simulink library "Scissor_Parts_Lib"  (R2025a)
settings: Solver=ode45  StartTime=0.0  StopTime=10.0  RelTol=1e-3  EnableMultiTasking=on
undefined symbols (not defined in the file or in its folder): Extr_Data_LinkHoles, Extr_Data_Ring, Local, Scissor_Lift_Param, X, Y, Z
libraries: sm_lib x23, $bdroot x16
Description:
  | Copyright 2015-2025 The MathWorks, Inc.
settings Model: Creator=smiller  LastModifiedBy=smiller
settings SolverCC: AlgebraicLoopSolver=TrustRegion
settings DataIOCC: LimitDataPoints=on  SaveFormat=Array  SignalLoggingSaveFormat=ModelDataLogs  ReturnWorkspaceOutputs=off
settings OptimizationCC: ReuseModelBlockBuffer=off  ExpressionDepthLimit=2147483647.0  LifeSpan=inf
settings DebuggingCC: UnderspecifiedInitializationDetection=Classic  MergeDetectMultiDrivingBlocksExec=none  SolverPrmCheckMsg=warning  FcnCallInpInsideContextMsg=warning  UnconnectedInputMsg=warning  UnconnectedOutputMsg=warning  UnconnectedLineMsg=warning  AllowSymbolicDim=off  StateNameClashWarn=warning  PregeneratedLibrarySubsystemCodeDiagnostic=none  SFUnexpectedBacktrackingDiag=warning  SFNoUnconditionalDefaultTransitionDiag=warning  SFExecutionAtInitializationDiag=none  ArithmeticOperatorsInVariantConditions=warning
settings HardwareCC: ProdBitPerPointer=32.0  ProdBitPerSizeT=32.0  ProdBitPerPtrDiffT=32.0  ProdLargestAtomicFloat=None  ProdIntDivRoundTo=Undefined  ProdEndianess=Unspecified  ProdWordSize=32.0  ProdHWDeviceType=32-bit Generic
settings ModelReferenceCC: EnableRefExpFcnMdlSchedulingChecks=on  PropagateSignalLabelsOutOfModel=off
settings SFSimCC: SimUseLocalCustomCode=off  CustomCodeUndefinedFunction=UseInterfaceOnly
settings RTWCC: RTWUseLocalCustomCode=off  GPUComputeCapability=3.5  DLArmComputeVersion=19.05
settings CodeAppCC: StateflowObjectComments=on
settings GRTTargetCC: TargetLangStandard=C89/C90 (ANSI)
settings ConfigComp: CovMetricSettings=dw  CovSaveCumulativeToWorkspaceVar=on  CovSaveSingleToWorkspaceVar=on  CovExternalEMLEnable=off  CovSFcnEnable=off

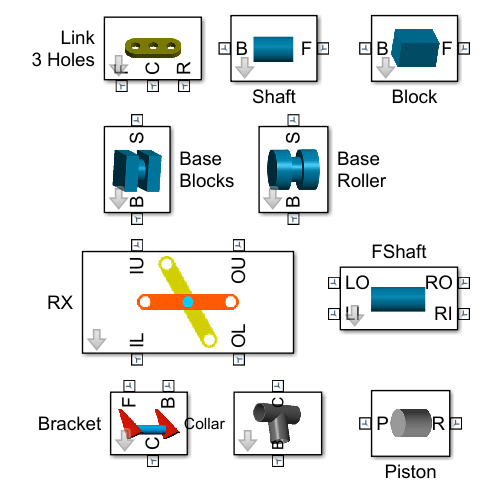
[thumbnail: Simulink's stored preview of the top-level diagram]
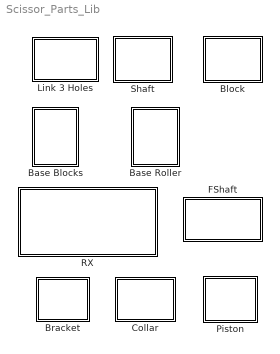
== system Scissor_Parts_Lib ==
  Base Blocks : Subsystem  mask(Base Blocks){block_length=Scissor_Lift_Param.Base_Block.Length, block_width=Scissor_Lift_Param.Base_Block.Width, block_height=Scissor_Lift_Param.Base_Block.Height, shaft_radius=Scissor_Lift_Param.Roller.Shaft_Radius, shaft_length=Scissor_Lift_Param.Roller.Shaft_Length, material_density=Scissor_Lift_Param.Base_Block.Density, material_color=Scissor_Lift_Param.Base_Block.Color, material_opacity=Scissor_Lift_Param.Base_Block.Opacity}
      mask prompts: block_length "Length (cm)"; block_width "Width (cm)"; block_height "Height (cm)"; shaft_radius "Radius (cm)"; shaft_length "Length (cm)"; material_density "Density (kg/m^3)"; material_color "Color"; material_opacity "Opacity"
      mask help: Parameterized base with two blocks and a shaft.
      mask Display:
      | image(imread('Base_Blocks_IMAGE.jpg'));
      | port_label('RConn',1,'S');
      | port_label('LConn',1,'B');
  Base Roller : Subsystem  mask(Base Roller){roller_length=Scissor_Lift_Param.Roller.Roller_Length, roller_radius=Scissor_Lift_Param.Roller.Roller_Radius, shaft_length=Scissor_Lift_Param.Roller.Shaft_Length, shaft_radius=Scissor_Lift_Param.Roller.Shaft_Radius, material_density=Scissor_Lift_Param.Roller.Density, material_color=Scissor_Lift_Param.Roller.Color, material_opacity=Scissor_Lift_Param.Roller.Opacity}
      mask prompts: roller_length "Length (cm)"; roller_radius "Radius (cm)"; shaft_length "Length (cm)"; shaft_radius "Radius (cm)"; material_density "Density (kg/m^3)"; material_color "Color"; material_opacity "Opacity"
      mask help: Parameterized roller with two wheels connected by a shaft.
      mask Display:
      | image(imread('Base_Roller_IMAGE.jpg'));
      | port_label('RConn',1,'S');
      | port_label('LConn',1,'B');
  Block : Subsystem  mask(Block){L=Scissor_Lift_Param.Base_Block.Length, W=Scissor_Lift_Param.Base_Block.Width, H=Scissor_Lift_Param.Base_Block.Height, z_ori=Local +Z, rho=Scissor_Lift_Param.Base_Block.Density, clr=Scissor_Lift_Param.Base_Block.Color, opc=Scissor_Lift_Param.Base_Block.Opacity}
      mask prompts: L "Length (cm):"; W "Width (cm):"; H "Height (cm):"; z_ori "Shaft orientation:"; rho "Shaft density (kg/m^3):"; clr "Link color:"; opc "Opacity:"
      mask help: Rectangular block. Ports are at the center of the faces normal to the local z-axis. Can be configured to have positive Z from B to F or from F to B.
      mask init:
      | if(z_ori == 2)
      |     z_ori = -1;
      | end
      mask TypeOptions z_ori: Local +Z | Local -Z
      mask DialogControl ParameterTabVar0 Prompt: Dimensions
      mask DialogControl ParameterTabVar01 Prompt: Material
      mask Display:
      | image(imread('Block_IMAGE.jpg'));
      | port_label('LConn',1,'B');
      | port_label('RConn',1,'F');
  Bracket : Subsystem  mask(Actuation Bracket){fl_w=Scissor_Lift_Param.Actuator.Bracket.Flange.Width, fl_h=Scissor_Lift_Param.Actuator.Bracket.Flange.Height, T=Scissor_Lift_Param.Actuator.Bracket.Flange.Thickness, W=Scissor_Lift_Param.Actuator.Bracket.Flange.Offset, flupdown=Down, flfrontrear=Rear, fl_density=Scissor_Lift_Param.Actuator.Bracket.Flange.Density, fl_clr=Scissor_Lift_Param.Actuator.Bracket.Flange.Color, fl_opc=Scissor_Lift_Param.Actuator.Bracket.Flange.Opacity, shaft_length=Scissor_Lift_Param.Link_Separation.Outer_Outer-Scissor_Lift_Param.Link_Separation.Outer_Inner*2, shaft_radius=Scissor_Lift_Param.Actuator.Bracket.Shaft.Radius, shaft_density=Scissor_Lift_Param.Actuator.Bracket.Shaft.Density, shaft_color=Scissor_Lift_Param.Actuator.Bracket.Shaft.Color, shaft_opacity=Scissor_Lift_Param.Actuator.Bracket.Shaft.Opacity}
      mask prompts: fl_w "Width (cm)"; fl_h "Height (cm)"; T "Thickness (cm)"; W "Offset (cm)"; flupdown "Orientation"; flfrontrear "Position"; fl_density "Density"; fl_clr "Color"; fl_opc "Opacity"; shaft_length "Length (cm)"; shaft_radius "Radius (cm)"; shaft_density "Density (kg/m^3)"; shaft_color "Color"; shaft_opacity "Opacity"
      mask help: Actuation bracket for scissor lift mechanism. Contains flanges that attach to links and connection shaft. Configurable orientation and surface attachment.
      mask init:
      | if(flupdown == 2)
      |     flupdown = -1;
      | end
      | if(flfrontrear == 2)
      |     flfrontrear = -1;
      | end
      mask TypeOptions flupdown: Up | Down
      mask TypeOptions flfrontrear: Front | Rear
      mask Display:
      | image(imread('Bracket_IMAGE.jpg'));
      | port_label('RConn',1,'F');
      | port_label('RConn',2,'B');
      | port_label('LConn',1,'C');
  Collar : Subsystem  mask{collar_length=Scissor_Lift_Param.Actuator.Collar.Length, collar_radius=Scissor_Lift_Param.Actuator.Collar.Radius, cylinder_length=Scissor_Lift_Param.Actuator.Piston_Seat.Length*2, cylinder_radius=Scissor_Lift_Param.Actuator.Piston_Seat.Radius, cylinder_ori=Local +Z, material_density=Scissor_Lift_Param.Actuator.Collar.Density, material_color=Scissor_Lift_Param.Actuator.Collar.Color, material_opacity=Scissor_Lift_Param.Actuator.Collar.Opacity}
      mask prompts: collar_length "Length (cm):"; collar_radius "Radius (cm):"; cylinder_length "Length (cm):"; cylinder_radius "Radius (cm):"; cylinder_ori "Orientation (B to C):"; material_density "Density (kg/m^3):"; material_color "Color:"; material_opacity "Opacity:"
      mask init:
      | if(cylinder_ori == 2)
      |     cylinder_ori = -1;
      | end
      mask TypeOptions cylinder_ori: Local +Z | Local -Z
      mask Display:
      | image(imread('Actuator_Collar_IMAGE.jpg'));
      | port_label('LConn',1,'B');
      | port_label('RConn',1,'C');
  FShaft : Subsystem  mask(Transverse Shaft){sep_outer_outer=Scissor_Lift_Param.Link_Separation.Outer_Outer, sep_outer_inner=Scissor_Lift_Param.Link_Separation.Outer_Inner, shaft_radius=Scissor_Lift_Param.Trans_Shaft.Radius, shaft_density=Scissor_Lift_Param.Trans_Shaft.Density, shaft_color=Scissor_Lift_Param.Trans_Shaft.Color, shaft_opacity=Scissor_Lift_Param.Trans_Shaft.Opacity}
      mask prompts: sep_outer_outer "Outer connection separation (cm)"; sep_outer_inner "Outer to inner separation (cm)"; shaft_radius "Radius (cm)"; shaft_density "Density (kg/m^3)"; shaft_color "Color"; shaft_opacity "Opacity"
      mask help: Transverse shaft with four connections. Frames are located at shaft center, with Z-axis along center.
      mask Display:
      | image(imread('Shaft_IMAGE.jpg'));
      | port_label('LConn',1,'LO');
      | port_label('LConn',2,'LI');
      | port_label('RConn',1,'RO');
      | port_label('RConn',2,'RI');
  Link 3 Holes : Subsystem  mask(Connector Link, 2 Holes){L=240, W=15, T=4, r=5, rho=1000, clr_string=Yellow, opc=1}
      mask prompts: L "Link length (cm):"; W "Link width (cm):"; T "Link thickness (cm):"; r "Hole radius (cm):"; rho "Link density (kg/m^3):"; clr_string "Link color:"; opc "Opacity:"
      mask help: Connector link with two holes. Ports are located at centers of holes, oriented such that Z is out of the hole, positive X is from L hole to R hole.
      mask init:
      | imgfile='Link_3_Hole_Yellow_IMAGE.jpg';
      | if(strcmp(clr_string,'Yellow'))
      |     clr = [0.6 0.6 0.0];
      | else
      |     clr = [0.8 0.2 0.0];
      |     imgfile='Link_3_Hole_Red_IMAGE.jpg';
      | end
      mask TypeOptions clr_string: Yellow | Red
      mask DialogControl ParameterTabVar0 Prompt: Dimensions
      mask DialogControl ParameterTabVar01 Prompt: Material
      mask Display:
      | image(imread(imgfile));
      | port_label('RConn',1,'F');
      | port_label('RConn',2,'C');
      | port_label('RConn',3,'R');
  Piston : Subsystem
      mask Display:
      | image(imread('Piston_Shaft_IMAGE.jpg'));
      | port_label('RConn',1,'P');
      | port_label('LConn',1,'R');
  RX : Subsystem  mask(Scissor Lift Crossbar){link_length=Scissor_Lift_Param.Link.Length, link_width=Scissor_Lift_Param.Link.Width, link_thickness=Scissor_Lift_Param.Link.Thickness, link_hole_radius=Scissor_Lift_Param.Link.Hole_Radius, link_density=Scissor_Lift_Param.Link.Density, link_color=Scissor_Lift_Param.Link.Color, link_opacity=Scissor_Lift_Param.Link.Opacity, shaft_length=Scissor_Lift_Param.Link_Separation.Outer_Inner, shaft_radius=Scissor_Lift_Param.Link_Pin.Radius, shaft_density=Scissor_Lift_Param.Link_Pin.Density, shaft_color=Scissor_Lift_Param.Link_Pin.Color, shaft_opacity=Scissor_Lift_Param.Link_Pin.Opacity, leftright=Right, imgfile=Crossbar_RX_IMAGE.jpg, L1Port=OU, L2Port=IU, R1Port=OL, R2Port=IL}
      mask prompts: link_length "Length (cm)"; link_width "Width (cm)"; link_thickness "Thickness (cm)"; link_hole_radius "Hole Radius (cm)"; link_density "Density (kg/m^3)"; link_color "Color"; link_opacity "Opacity"; shaft_length "Length (cm)"; shaft_radius "Radius (cm)"; shaft_density "Density (kg/m^3)"; shaft_color "Color"; shaft_opacity "Opacity"; leftright "Side"; imgfile "Image File"; L1Port "L1 Port Name"; L2Port "L2 Port Name"; R1Port "R1 Port Name"; R2Port "R2 Port Name"
      mask help: Parameterized crossbar. The two links are connected by a revolute joint. Configurable for left or right side.
      mask init:
      | pinbpth = find_system(gcb,'MatchFilter',@Simulink.match.allVariants,'LookUnderMasks','on','FollowLinks','on','Regexp','on','BlockDialogParams','^Local');
      | %get_param(pinbpth,'z_ori')
      | %leftright
      | %if(1==2)
      | if (leftright == 1)
      |     %disp('Setting to 0, LEFT');
      |     set_param(char(pinbpth),'z_ori',1);
      |     set_param([gcb '/OL'],'Port','1','Side','Right');
      |     set_param([gcb '/IL'],'Port','2','Side','Right');
      |     set_param([gcb '/OU'],'Port','3','Side','Left');
      |     set_param([gcb '/IU'],'Port','4','Side','Left');
      |     set_param(gcb,'Name','LX');
      |     L1Port='OU';
      |     L2Port='IU';
      |     R1Port='OL';
      |     R2Port='IL';
      |     imgfile = 'Crossbar_LX_IMAGE.jpg';
      | else
      |     %disp('Setting to 1, RIGHT');
      |     set_param(char(pinbpth),'z_ori',0);
      |     set_param([gcb '/IL'],'Port','1','Side','Right');
      |     set_param([gcb '/OL'],'Port','2','Side','Right');
      |     set_param([gcb '/IU'],'Port','3','Side','Left');
      |     set_param([gcb '/OU'],'Port','4','Side','Left');
      |     set_param(gcb,'Name','RX');
      |     L1Port='IU';
      |     L2Port='OU';
      |     R1Port='IL';
      |     R2Port='OL';
      |     imgfile = 'Crossbar_RX_IMAGE.jpg';
      | end
      | %end
      mask TypeOptions leftright: Left | Right
      mask DialogControl ParameterTabVar0 Prompt: Links
      mask DialogControl ParameterTabVar01 Prompt: Shaft
      mask Display:
      | image(imread(imgfile));
      | port_label('LConn',1,L1Port);
      | port_label('LConn',2,L2Port);
      | port_label('RConn',1,R1Port);
      | port_label('RConn',2,R2Port);
  Shaft : Subsystem  mask(Cylindrical Shaft){L=10, r=5, theta=0, z_ori=Local -Z, Ro=1000, clr=[0.0 0.6 0.8], opc=1}
      mask prompts: L "Length (cm):"; r "Radius (cm):"; theta "Twist (deg)"; z_ori "Orientation (B to F)"; Ro "Density (kg/m^3):"; clr "Color:"; opc "Opacity"
      mask help: Cylindrical shaft. Ports are at shaft ends, and oriented such that the Z-axis is between the ports. Can be configured to have positive Z from B to F or from F to B.
      mask init:
      | if(z_ori == 2)
      |     z_ori = -1;
      | end
      mask TypeOptions z_ori: Local +Z | Local -Z
      mask Display:
      | image(imread('Shaft_IMAGE.jpg'));
      | port_label('LConn',1,'B');
      | port_label('RConn',1,'F');

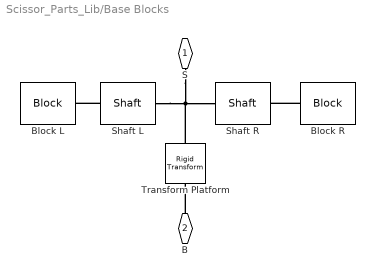
== system Scissor_Parts_Lib/Base Blocks ==
  Block L : $bdroot/Block  L=block_length  W=block_width  H=block_height  z_ori=Local -Z  rho=material_density  clr=material_color  opc=material_opacity
  Block R : $bdroot/Block  L=block_length  W=block_width  H=block_height  z_ori=Local +Z  rho=material_density  clr=material_color  opc=material_opacity
  Shaft L : $bdroot/Shaft  L=shaft_length/2  r=shaft_radius  theta=0  z_ori=Local -Z  Ro=material_density  clr=material_color  opc=material_opacity
  Shaft R : $bdroot/Shaft  L=shaft_length/2  r=shaft_radius  theta=0  z_ori=Local +Z  Ro=material_density  clr=material_color  opc=material_opacity
  Transform Platform : sm_lib/Frames and Transforms/Rigid Transform  RotationMethod=None  FollAlignAxisA=+X  BaseAlignAxisA=+Y  FollAlignAxisB=+Y  BaseAlignAxisB=+Z  RotationStandardAxis=+Y  RotationAngle=0  RotationAngleUnits=deg  RotationArbitraryAxis=[0 0 1]  RotationSequenceAxes=FollowerAxes  RotationSequence=XYX  RotationSequenceAngles=[0 0 0]  RotationSequenceAnglesUnits=deg  RotationMatrix=[1 0 0; 0 1 0; 0 0 1]  Quaternion=[1 0 0 0]  TranslationMethod=Cartesian  TranslationCartesianOffset=[0 -block_height/2 0]  TranslationCartesianOffsetUnits=cm  TranslationStandardAxis=-Y  TranslationStandardOffset=Scissor_Lift_Param.Roller.Roller_Radius  TranslationStandardOffsetUnits=cm  TranslationROffset=0  TranslationROffsetUnits=m  TranslationThetaOffset=0  TranslationThetaOffsetUnits=deg  TranslationZOffset=0  TranslationZOffsetUnits=m
  S : PMIOPort  Side=Right
  B : PMIOPort  Port=2  Side=Left
  connections:
  Shaft L/RConn1 -- Block L/LConn1
  Block R/LConn1 -- Shaft R/RConn1
  B/RConn1 -- Transform Platform/RConn1
  Shaft L/LConn1 -- Shaft R/LConn1 -- Transform Platform/LConn1 -- S/RConn1

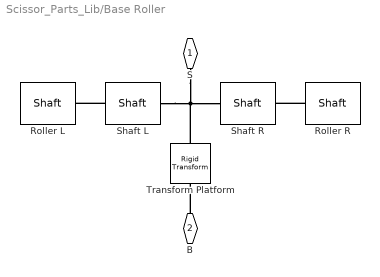
== system Scissor_Parts_Lib/Base Roller ==
  Roller L : $bdroot/Shaft  L=roller_length  r=roller_radius  theta=0  z_ori=Local -Z  Ro=material_density  clr=material_color  opc=material_opacity
  Roller R : $bdroot/Shaft  L=roller_length  r=roller_radius  theta=0  z_ori=Local +Z  Ro=material_density  clr=material_color  opc=material_opacity
  Shaft L : $bdroot/Shaft  L=shaft_length/2  r=shaft_radius  theta=0  z_ori=Local -Z  Ro=material_density  clr=material_color  opc=material_opacity
  Shaft R : $bdroot/Shaft  L=shaft_length/2  r=shaft_radius  theta=0  z_ori=Local +Z  Ro=material_density  clr=material_color  opc=material_opacity
  Transform Platform : sm_lib/Frames and Transforms/Rigid Transform  RotationMethod=StandardAxis  FollAlignAxisA=+X  BaseAlignAxisA=+Y  FollAlignAxisB=+Y  BaseAlignAxisB=+Z  RotationStandardAxis=+Y  RotationAngle=90  RotationAngleUnits=deg  RotationArbitraryAxis=[0 0 1]  RotationSequenceAxes=FollowerAxes  RotationSequence=XYX  RotationSequenceAngles=[0 0 0]  RotationSequenceAnglesUnits=deg  RotationMatrix=[1 0 0; 0 1 0; 0 0 1]  Quaternion=[1 0 0 0]  TranslationMethod=StandardAxis  TranslationCartesianOffset=[0 0 0]  TranslationCartesianOffsetUnits=cm  TranslationStandardAxis=-Y  TranslationStandardOffset=roller_radius  TranslationStandardOffsetUnits=cm  TranslationROffset=0  TranslationROffsetUnits=m  TranslationThetaOffset=0  TranslationThetaOffsetUnits=deg  TranslationZOffset=0  TranslationZOffsetUnits=m
  S : PMIOPort  Side=Right
  B : PMIOPort  Port=2  Side=Left
  connections:
  Shaft L/RConn1 -- Roller L/LConn1
  Roller R/LConn1 -- Shaft R/RConn1
  S/RConn1 -- Shaft L/LConn1 -- Transform Platform/LConn1 -- Shaft R/LConn1
  B/RConn1 -- Transform Platform/RConn1

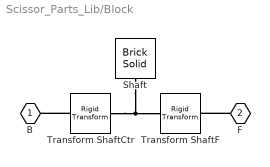
== system Scissor_Parts_Lib/Block ==
  Shaft : sm_lib/Body Elements/Brick Solid  BrickDimensions=[W H L]  BrickDimensionsUnits=cm  ExportEntireGeometry=off  InertiaType=CalculateFromGeometry  BasedOnType=Density  Density=rho  DensityUnits=kg/m^3  Mass=1  MassUnits=kg  CenterOfMass=[0 0 0]  CenterOfMassUnits=m  MomentsOfInertia=[1 1 1]  MomentsOfInertiaUnits=kg*m^2  ProductsOfInertia=[0 0 0]  ProductsOfInertiaUnits=kg*m^2  GraphicType=FromGeometry  MarkerShape=Sphere  MarkerSize=1  GraphicVisPropType=SimpleVisualProperties  GraphicDiffuseColor=clr  GraphicOpacity=opc  GraphicSpecularColor=[0.2 0.2 0.2]  GraphicAmbientColor=[0.5 0.5 0.5]  GraphicEmissiveColor=[0.1 0.1 0.1]  GraphicShininess=24.0  DoExposeReferenceFrame=on  SerializedFrames=<Frames/>
  Transform ShaftCtr : sm_lib/Frames and Transforms/Rigid Transform  RotationMethod=None  FollAlignAxisA=+X  BaseAlignAxisA=+Y  FollAlignAxisB=+Y  BaseAlignAxisB=+Z  RotationStandardAxis=+Z  RotationAngle=0  RotationAngleUnits=deg  RotationArbitraryAxis=[0 0 1]  RotationSequenceAxes=FollowerAxes  RotationSequence=XYX  RotationSequenceAngles=[0 0 0]  RotationSequenceAnglesUnits=deg  RotationMatrix=[1 0 0; 0 1 0; 0 0 1]  Quaternion=[1 0 0 0]  TranslationMethod=Cartesian  TranslationCartesianOffset=[0 0 L/2]*z_ori  TranslationCartesianOffsetUnits=cm  TranslationStandardAxis=+Z  TranslationStandardOffset=0  TranslationStandardOffsetUnits=cm  TranslationROffset=0  TranslationROffsetUnits=m  TranslationThetaOffset=0  TranslationThetaOffsetUnits=deg  TranslationZOffset=0  TranslationZOffsetUnits=m
  Transform ShaftF : sm_lib/Frames and Transforms/Rigid Transform  RotationMethod=None  FollAlignAxisA=+X  BaseAlignAxisA=+Y  FollAlignAxisB=+Y  BaseAlignAxisB=+Z  RotationStandardAxis=+Z  RotationAngle=0  RotationAngleUnits=deg  RotationArbitraryAxis=[0 0 1]  RotationSequenceAxes=FollowerAxes  RotationSequence=XYX  RotationSequenceAngles=[0 0 0]  RotationSequenceAnglesUnits=deg  RotationMatrix=[1 0 0; 0 1 0; 0 0 1]  Quaternion=[1 0 0 0]  TranslationMethod=Cartesian  TranslationCartesianOffset=[0 0 L/2]*z_ori  TranslationCartesianOffsetUnits=cm  TranslationStandardAxis=+Z  TranslationStandardOffset=0  TranslationStandardOffsetUnits=cm  TranslationROffset=0  TranslationROffsetUnits=m  TranslationThetaOffset=0  TranslationThetaOffsetUnits=deg  TranslationZOffset=0  TranslationZOffsetUnits=m
  B : PMIOPort  Side=Left
  F : PMIOPort  Port=2  Side=Right
  connections:
  Transform ShaftCtr/LConn1 -- B/RConn1
  F/RConn1 -- Transform ShaftF/RConn1
  Shaft/RConn1 -- Transform ShaftF/LConn1 -- Transform ShaftCtr/RConn1

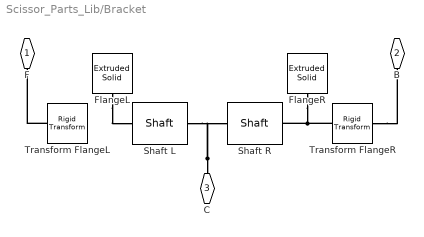
== system Scissor_Parts_Lib/Bracket ==
  FlangeL : sm_lib/Body Elements/Extruded Solid  ExtrusionType=General  PolygonNumSides=1  PolygonOuterRadius=1  PolygonOuterRadiusUnits=m  ExportEntireGeometry=off  ExtrusionCrossSection=[0 fl_h;-fl_w -fl_h;fl_w -fl_h]*0.5*flupdown  ExtrusionCrossSectionUnits=cm  ExportConvexHullGeometry=off  ExtrusionLength=T  ExtrusionLengthUnits=cm  InertiaType=CalculateFromGeometry  BasedOnType=Density  Density=fl_density  DensityUnits=kg/m^3  Mass=1  MassUnits=kg  CenterOfMass=[0 0 0]  CenterOfMassUnits=m  MomentsOfInertia=[1 1 1]  MomentsOfInertiaUnits=kg*m^2  ProductsOfInertia=[0 0 0]  ProductsOfInertiaUnits=kg*m^2  GraphicType=FromGeometry  MarkerShape=Sphere  MarkerSize=1  GraphicVisPropType=SimpleVisualProperties  GraphicDiffuseColor=fl_clr  GraphicOpacity=fl_opc  GraphicSpecularColor=[0.2 0.2 0.2]  GraphicAmbientColor=[0.5 0.5 0.5]  GraphicEmissiveColor=[0.1 0.1 0.1]  GraphicShininess=24.0  DoExposeReferenceFrame=on  SerializedFrames=<Frames/>
  FlangeR : sm_lib/Body Elements/Extruded Solid  ExtrusionType=General  PolygonNumSides=1  PolygonOuterRadius=1  PolygonOuterRadiusUnits=m  ExportEntireGeometry=off  ExtrusionCrossSection=[0 fl_h;-fl_w -fl_h;fl_w -fl_h]*0.5*flupdown  ExtrusionCrossSectionUnits=cm  ExportConvexHullGeometry=off  ExtrusionLength=T  ExtrusionLengthUnits=cm  InertiaType=CalculateFromGeometry  BasedOnType=Density  Density=fl_density  DensityUnits=kg/m^3  Mass=1  MassUnits=kg  CenterOfMass=[0 0 0]  CenterOfMassUnits=m  MomentsOfInertia=[1 1 1]  MomentsOfInertiaUnits=kg*m^2  ProductsOfInertia=[0 0 0]  ProductsOfInertiaUnits=kg*m^2  GraphicType=FromGeometry  MarkerShape=Sphere  MarkerSize=1  GraphicVisPropType=SimpleVisualProperties  GraphicDiffuseColor=fl_clr  GraphicOpacity=fl_opc  GraphicSpecularColor=[0.2 0.2 0.2]  GraphicAmbientColor=[0.5 0.5 0.5]  GraphicEmissiveColor=[0.1 0.1 0.1]  GraphicShininess=24.0  DoExposeReferenceFrame=on  SerializedFrames=<Frames/>
  Shaft L : $bdroot/Shaft  L=shaft_length/2  r=shaft_radius  theta=0  z_ori=Local -Z  Ro=shaft_density  clr=shaft_color  opc=shaft_opacity
  Shaft R : $bdroot/Shaft  L=shaft_length/2  r=shaft_radius  theta=0  z_ori=Local -Z  Ro=shaft_density  clr=shaft_color  opc=shaft_opacity
  Transform FlangeL : sm_lib/Frames and Transforms/Rigid Transform  RotationMethod=None  FollAlignAxisA=+X  BaseAlignAxisA=+Y  FollAlignAxisB=+Y  BaseAlignAxisB=+Z  RotationStandardAxis=+Z  RotationAngle=0  RotationAngleUnits=deg  RotationArbitraryAxis=[0 0 1]  RotationSequenceAxes=FollowerAxes  RotationSequence=XYX  RotationSequenceAngles=[0 0 0]  RotationSequenceAnglesUnits=deg  RotationMatrix=[1 0 0; 0 1 0; 0 0 1]  Quaternion=[1 0 0 0]  TranslationMethod=Cartesian  TranslationCartesianOffset=[(fl_w/2)*flfrontrear (fl_h/2+W/2)*flupdown 0]  TranslationCartesianOffsetUnits=cm  TranslationStandardAxis=-X  TranslationStandardOffset=1  TranslationStandardOffsetUnits=cm  TranslationROffset=0  TranslationROffsetUnits=m  TranslationThetaOffset=0  TranslationThetaOffsetUnits=deg  TranslationZOffset=0  TranslationZOffsetUnits=m
  Transform FlangeR : sm_lib/Frames and Transforms/Rigid Transform  RotationMethod=None  FollAlignAxisA=+X  BaseAlignAxisA=+Y  FollAlignAxisB=+Y  BaseAlignAxisB=+Z  RotationStandardAxis=+Z  RotationAngle=0  RotationAngleUnits=deg  RotationArbitraryAxis=[0 0 1]  RotationSequenceAxes=FollowerAxes  RotationSequence=XYX  RotationSequenceAngles=[0 0 0]  RotationSequenceAnglesUnits=deg  RotationMatrix=[1 0 0; 0 1 0; 0 0 1]  Quaternion=[1 0 0 0]  TranslationMethod=Cartesian  TranslationCartesianOffset=[(fl_w/2)*flfrontrear (fl_h/2+W/2)*flupdown 0]  TranslationCartesianOffsetUnits=cm  TranslationStandardAxis=-X  TranslationStandardOffset=1  TranslationStandardOffsetUnits=cm  TranslationROffset=0  TranslationROffsetUnits=m  TranslationThetaOffset=0  TranslationThetaOffsetUnits=deg  TranslationZOffset=0  TranslationZOffsetUnits=m
  F : PMIOPort  Side=Right
  B : PMIOPort  Port=2  Side=Right
  C : PMIOPort  Port=3  Side=Left
  connections:
  Transform FlangeL/LConn1 -- F/RConn1
  Transform FlangeR/LConn1 -- B/RConn1
  FlangeR/RConn1 -- Shaft R/RConn1 -- Transform FlangeR/RConn1
  FlangeL/RConn1 -- Shaft L/LConn1
  C/RConn1 -- Shaft L/RConn1 -- Shaft R/LConn1

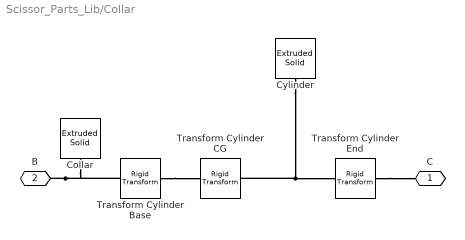
== system Scissor_Parts_Lib/Collar ==
  Collar : sm_lib/Body Elements/Extruded Solid  ExtrusionType=General  PolygonNumSides=3  PolygonOuterRadius=1  PolygonOuterRadiusUnits=m  ExportEntireGeometry=off  ExtrusionCrossSection=Extr_Data_Ring(collar_radius,collar_radius*0.9,0,360)  ExtrusionCrossSectionUnits=cm  ExportConvexHullGeometry=off  ExtrusionLength=collar_length  ExtrusionLengthUnits=cm  InertiaType=CalculateFromGeometry  BasedOnType=Density  Density=material_density  DensityUnits=kg/(m^3)  Mass=1  MassUnits=kg  CenterOfMass=[0 0 0]  CenterOfMassUnits=m  MomentsOfInertia=[1 1 1]  MomentsOfInertiaUnits=kg*m^2  ProductsOfInertia=[0 0 0]  ProductsOfInertiaUnits=kg*m^2  GraphicType=FromGeometry  MarkerShape=Sphere  MarkerSize=10  GraphicVisPropType=SimpleVisualProperties  GraphicDiffuseColor=material_color  GraphicOpacity=material_opacity  GraphicSpecularColor=[0.5 0.5 0.5 1.0]  GraphicAmbientColor=[0.15 0.15 0.15 1.0]  GraphicEmissiveColor=[0.0 0.0 0.0 1.0]  GraphicShininess=75  DoExposeReferenceFrame=on  SerializedFrames=<Frames/>
  Cylinder : sm_lib/Body Elements/Extruded Solid  ExtrusionType=General  PolygonNumSides=3  PolygonOuterRadius=1  PolygonOuterRadiusUnits=m  ExportEntireGeometry=off  ExtrusionCrossSection=Extr_Data_Ring(cylinder_radius,cylinder_radius*0.9,0,360)  ExtrusionCrossSectionUnits=cm  ExportConvexHullGeometry=off  ExtrusionLength=cylinder_length  ExtrusionLengthUnits=cm  InertiaType=CalculateFromGeometry  BasedOnType=Density  Density=material_density  DensityUnits=kg/(m^3)  Mass=1  MassUnits=kg  CenterOfMass=[0 0 0]  CenterOfMassUnits=m  MomentsOfInertia=[1 1 1]  MomentsOfInertiaUnits=kg*m^2  ProductsOfInertia=[0 0 0]  ProductsOfInertiaUnits=kg*m^2  GraphicType=FromGeometry  MarkerShape=Sphere  MarkerSize=10  GraphicVisPropType=SimpleVisualProperties  GraphicDiffuseColor=material_color  GraphicOpacity=material_opacity  GraphicSpecularColor=[0.5 0.5 0.5 1.0]  GraphicAmbientColor=[0.15 0.15 0.15 1.0]  GraphicEmissiveColor=[0.0 0.0 0.0 1.0]  GraphicShininess=75  DoExposeReferenceFrame=on  SerializedFrames=<Frames/>
  Transform Cylinder Base : sm_lib/Frames and Transforms/Rigid Transform  RotationMethod=StandardAxis  FollAlignAxisA=+X  BaseAlignAxisA=+Y  FollAlignAxisB=+Y  BaseAlignAxisB=+Z  RotationStandardAxis=-Y  RotationAngle=90  RotationAngleUnits=deg  RotationArbitraryAxis=[0 0 1]  RotationSequenceAxes=FollowerAxes  RotationSequence=XYX  RotationSequenceAngles=[0 0 0]  RotationSequenceAnglesUnits=deg  RotationMatrix=[1 0 0; 0 1 0; 0 0 1]  Quaternion=[1 0 0 0]  TranslationMethod=None  TranslationCartesianOffset=[0 0 0]  TranslationCartesianOffsetUnits=m  TranslationStandardAxis=+Z  TranslationStandardOffset=0  TranslationStandardOffsetUnits=m  TranslationROffset=0  TranslationROffsetUnits=m  TranslationThetaOffset=0  TranslationThetaOffsetUnits=deg  TranslationZOffset=0  TranslationZOffsetUnits=m
  Transform Cylinder CG : sm_lib/Frames and Transforms/Rigid Transform  RotationMethod=None  FollAlignAxisA=+X  BaseAlignAxisA=+Y  FollAlignAxisB=+Y  BaseAlignAxisB=+Z  RotationStandardAxis=+Y  RotationAngle=0  RotationAngleUnits=deg  RotationArbitraryAxis=[0 0 1]  RotationSequenceAxes=FollowerAxes  RotationSequence=XYX  RotationSequenceAngles=[0 0 0]  RotationSequenceAnglesUnits=deg  RotationMatrix=[1 0 0; 0 1 0; 0 0 1]  Quaternion=[1 0 0 0]  TranslationMethod=StandardAxis  TranslationCartesianOffset=[0 0 0]  TranslationCartesianOffsetUnits=cm  TranslationStandardAxis=+Z  TranslationStandardOffset=cylinder_length/2*cylinder_ori  TranslationStandardOffsetUnits=cm  TranslationROffset=0  TranslationROffsetUnits=m  TranslationThetaOffset=0  TranslationThetaOffsetUnits=deg  TranslationZOffset=0  TranslationZOffsetUnits=m
  Transform Cylinder End : sm_lib/Frames and Transforms/Rigid Transform  RotationMethod=None  FollAlignAxisA=+X  BaseAlignAxisA=+Y  FollAlignAxisB=+Y  BaseAlignAxisB=+Z  RotationStandardAxis=+Y  RotationAngle=0  RotationAngleUnits=deg  RotationArbitraryAxis=[0 0 1]  RotationSequenceAxes=FollowerAxes  RotationSequence=XYX  RotationSequenceAngles=[0 0 0]  RotationSequenceAnglesUnits=deg  RotationMatrix=[1 0 0; 0 1 0; 0 0 1]  Quaternion=[1 0 0 0]  TranslationMethod=StandardAxis  TranslationCartesianOffset=[0 0 0]  TranslationCartesianOffsetUnits=cm  TranslationStandardAxis=+Z  TranslationStandardOffset=cylinder_length/2*cylinder_ori  TranslationStandardOffsetUnits=cm  TranslationROffset=0  TranslationROffsetUnits=m  TranslationThetaOffset=0  TranslationThetaOffsetUnits=deg  TranslationZOffset=0  TranslationZOffsetUnits=m
  C : PMIOPort  Side=Right
  B : PMIOPort  Port=2  Side=Left
  connections:
  Transform Cylinder Base/RConn1 -- Transform Cylinder CG/LConn1
  Cylinder/RConn1 -- Transform Cylinder End/LConn1 -- Transform Cylinder CG/RConn1
  B/RConn1 -- Collar/RConn1 -- Transform Cylinder Base/LConn1
  Transform Cylinder End/RConn1 -- C/RConn1

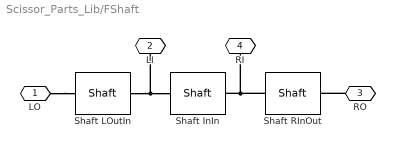
== system Scissor_Parts_Lib/FShaft ==
  Shaft InIn : $bdroot/Shaft  L=sep_outer_outer-2*sep_outer_inner  r=shaft_radius  theta=0  z_ori=Local -Z  Ro=shaft_density  clr=shaft_color  opc=shaft_opacity
  Shaft LOutIn : $bdroot/Shaft  L=sep_outer_inner  r=shaft_radius  theta=0  z_ori=Local -Z  Ro=shaft_density  clr=shaft_color  opc=shaft_opacity
  Shaft RInOut : $bdroot/Shaft  L=sep_outer_inner  r=shaft_radius  theta=0  z_ori=Local -Z  Ro=shaft_density  clr=shaft_color  opc=shaft_opacity
  LO : PMIOPort  Side=Left
  LI : PMIOPort  Port=2  Side=Left
  RO : PMIOPort  Port=3  Side=Right
  RI : PMIOPort  Port=4  Side=Right
  connections:
  Shaft LOutIn/RConn1 -- LI/RConn1 -- Shaft InIn/LConn1
  Shaft RInOut/LConn1 -- Shaft InIn/RConn1 -- RI/RConn1
  LO/RConn1 -- Shaft LOutIn/LConn1
  RO/RConn1 -- Shaft RInOut/RConn1

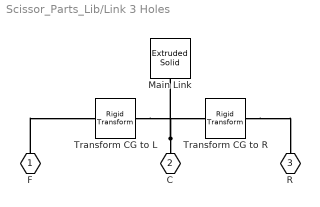
== system Scissor_Parts_Lib/Link 3 Holes ==
  Main Link : sm_lib/Body Elements/Extruded Solid  ExtrusionType=General  PolygonNumSides=1  PolygonOuterRadius=1  PolygonOuterRadiusUnits=m  ExportEntireGeometry=off  ExtrusionCrossSection=Extr_Data_LinkHoles(L,W,r,3)  ExtrusionCrossSectionUnits=cm  ExportConvexHullGeometry=off  ExtrusionLength=T  ExtrusionLengthUnits=cm  InertiaType=CalculateFromGeometry  BasedOnType=Density  Density=rho  DensityUnits=kg/m^3  Mass=1  MassUnits=kg  CenterOfMass=[0 0 0]  CenterOfMassUnits=m  MomentsOfInertia=[1 1 1]  MomentsOfInertiaUnits=kg*m^2  ProductsOfInertia=[0 0 0]  ProductsOfInertiaUnits=kg*m^2  GraphicType=FromGeometry  MarkerShape=Sphere  MarkerSize=1  GraphicVisPropType=SimpleVisualProperties  GraphicDiffuseColor=clr  GraphicOpacity=opc  GraphicSpecularColor=[0.2 0.2 0.2]  GraphicAmbientColor=[0.5 0.5 0.5]  GraphicEmissiveColor=[0.1 0.1 0.1]  GraphicShininess=24.0  DoExposeReferenceFrame=on  SerializedFrames=<Frames/>
  Transform CG to L : sm_lib/Frames and Transforms/Rigid Transform  RotationMethod=None  FollAlignAxisA=+X  BaseAlignAxisA=+Y  FollAlignAxisB=+Y  BaseAlignAxisB=+Z  RotationStandardAxis=+Z  RotationAngle=0  RotationAngleUnits=deg  RotationArbitraryAxis=[0 0 1]  RotationSequenceAxes=FollowerAxes  RotationSequence=XYX  RotationSequenceAngles=[0 0 0]  RotationSequenceAnglesUnits=deg  RotationMatrix=[1 0 0; 0 1 0; 0 0 1]  Quaternion=[1 0 0 0]  TranslationMethod=StandardAxis  TranslationCartesianOffset=[0 0 0]  TranslationCartesianOffsetUnits=cm  TranslationStandardAxis=-X  TranslationStandardOffset=L/2  TranslationStandardOffsetUnits=cm  TranslationROffset=0  TranslationROffsetUnits=m  TranslationThetaOffset=0  TranslationThetaOffsetUnits=deg  TranslationZOffset=0  TranslationZOffsetUnits=m
  Transform CG to R : sm_lib/Frames and Transforms/Rigid Transform  RotationMethod=None  FollAlignAxisA=+X  BaseAlignAxisA=+Y  FollAlignAxisB=+Y  BaseAlignAxisB=+Z  RotationStandardAxis=+Z  RotationAngle=0  RotationAngleUnits=deg  RotationArbitraryAxis=[0 0 1]  RotationSequenceAxes=FollowerAxes  RotationSequence=XYX  RotationSequenceAngles=[0 0 0]  RotationSequenceAnglesUnits=deg  RotationMatrix=[1 0 0; 0 1 0; 0 0 1]  Quaternion=[1 0 0 0]  TranslationMethod=StandardAxis  TranslationCartesianOffset=[0 0 0]  TranslationCartesianOffsetUnits=cm  TranslationStandardAxis=+X  TranslationStandardOffset=L/2  TranslationStandardOffsetUnits=cm  TranslationROffset=0  TranslationROffsetUnits=m  TranslationThetaOffset=0  TranslationThetaOffsetUnits=deg  TranslationZOffset=0  TranslationZOffsetUnits=m
  F : PMIOPort  Side=Right
  C : PMIOPort  Port=2  Side=Right
  R : PMIOPort  Port=3  Side=Right
  connections:
  Transform CG to R/RConn1 -- R/RConn1
  C/RConn1 -- Transform CG to L/LConn1 -- Main Link/RConn1 -- Transform CG to R/LConn1
  F/RConn1 -- Transform CG to L/RConn1

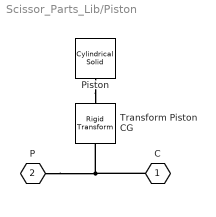
== system Scissor_Parts_Lib/Piston ==
  Piston : sm_lib/Body Elements/Cylindrical Solid  CylinderRadius=Scissor_Lift_Param.Actuator.Piston_Radius  CylinderRadiusUnits=cm  CylinderLength=Scissor_Lift_Param.Actuator.Piston_Length  CylinderLengthUnits=cm  ExportEntireGeometry=off  InertiaType=CalculateFromGeometry  BasedOnType=Density  Density=1000  DensityUnits=kg/(m^3)  Mass=1  MassUnits=kg  CenterOfMass=[0 0 0]  CenterOfMassUnits=m  MomentsOfInertia=[1 1 1]  MomentsOfInertiaUnits=kg*m^2  ProductsOfInertia=[0 0 0]  ProductsOfInertiaUnits=kg*m^2  GraphicType=FromGeometry  MarkerShape=Sphere  MarkerSize=10  GraphicVisPropType=SimpleVisualProperties  GraphicDiffuseColor=[0.8 0.8 0.8]  GraphicOpacity=1.0  GraphicSpecularColor=[0.5 0.5 0.5 1.0]  GraphicAmbientColor=[0.15 0.15 0.15 1.0]  GraphicEmissiveColor=[0.0 0.0 0.0 1.0]  GraphicShininess=75  DoExposeReferenceFrame=on  SerializedFrames=<Frames/>
  Transform Piston CG : sm_lib/Frames and Transforms/Rigid Transform  RotationMethod=None  FollAlignAxisA=+X  BaseAlignAxisA=+Y  FollAlignAxisB=+Y  BaseAlignAxisB=+Z  RotationStandardAxis=+Y  RotationAngle=0  RotationAngleUnits=deg  RotationArbitraryAxis=[0 0 1]  RotationSequenceAxes=FollowerAxes  RotationSequence=XYX  RotationSequenceAngles=[0 0 0]  RotationSequenceAnglesUnits=deg  RotationMatrix=[1 0 0; 0 1 0; 0 0 1]  Quaternion=[1 0 0 0]  TranslationMethod=StandardAxis  TranslationCartesianOffset=[0 0 0]  TranslationCartesianOffsetUnits=cm  TranslationStandardAxis=-Z  TranslationStandardOffset=Scissor_Lift_Param.Actuator.Piston_Length/2  TranslationStandardOffsetUnits=cm  TranslationROffset=0  TranslationROffsetUnits=m  TranslationThetaOffset=0  TranslationThetaOffsetUnits=deg  TranslationZOffset=0  TranslationZOffsetUnits=m
  C : PMIOPort  Side=Left
  P : PMIOPort  Port=2  Side=Right
  connections:
  Piston/RConn1 -- Transform Piston CG/RConn1
  C/RConn1 -- Transform Piston CG/LConn1 -- P/RConn1

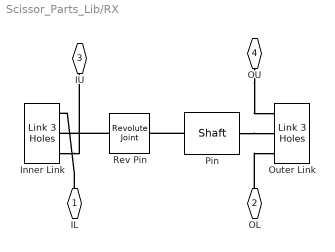
== system Scissor_Parts_Lib/RX ==
  Inner Link : $bdroot/Link 3 Holes  L=link_length  W=link_width  T=link_thickness  r=link_hole_radius  rho=link_density  clr_string=Red  opc=link_opacity
  Outer Link : $bdroot/Link 3 Holes  L=link_length  W=link_width  T=link_thickness  r=link_hole_radius  rho=link_density  clr_string=Yellow  opc=link_opacity
  Pin : $bdroot/Shaft  L=shaft_length  r=shaft_radius  theta=0  z_ori=Local +Z  Ro=shaft_density  clr=shaft_color  opc=shaft_opacity
  Rev Pin : sm_lib/Joints/Revolute Joint  JointMode=Normal  CompositeWrenchDir=FollowerOnBase  CompositeWrenchFrame=BaseFrame  SenseConstraintForce=off  SenseConstraintTorque=off  SenseTotalForce=off  SenseTotalTorque=off  PositionTargetSpecify=off  PositionTargetPriority=High  PositionTargetValue=0  PositionTargetValueUnits=rad  VelocityTargetSpecify=off  VelocityTargetPriority=High  VelocityTargetValue=0  VelocityTargetValueUnits=rad/s  EquilibriumPosition=0  EquilibriumPositionUnits=rad  SpringStiffness=0  SpringStiffnessUnits=N*m/rad  DampingCoefficient=0  DampingCoefficientUnits=N*m/(rad/s)  LowerLimitSpecify=off  LowerLimitBound=-90  LowerLimitBoundUnits=deg  LowerLimitStiffness=1e4  LowerLimitStiffnessUnits=N*m/deg  LowerLimitDamping=10  LowerLimitDampingUnits=N*m/(deg/s)  LowerLimitTransitionRegionWidth=0.1  LowerLimitTransitionRegionWidthUnits=deg  UpperLimitSpecify=off  UpperLimitBound=90  UpperLimitBoundUnits=deg  UpperLimitStiffness=1e4  UpperLimitStiffnessUnits=N*m/deg  UpperLimitDamping=10  UpperLimitDampingUnits=N*m/(deg/s)  UpperLimitTransitionRegionWidth=0.1  UpperLimitTransitionRegionWidthUnits=deg  TorqueActuationMode=NoTorque  MotionActuationMode=ComputedMotion  SensePosition=off  SenseVelocity=off  SenseAcceleration=off  SenseTorqueForce=off  SenseLowerLimitTorqueForce=off  SenseUpperLimitTorqueForce=off
  IL : PMIOPort  Side=Right
  OL : PMIOPort  Port=2  Side=Right
  IU : PMIOPort  Port=3  Side=Left
  OU : PMIOPort  Port=4  Side=Left
  connections:
  Inner Link/RConn3 -- IU/RConn1
  OL/RConn1 -- Outer Link/RConn3
  IL/RConn1 -- Inner Link/RConn1
  OU/RConn1 -- Outer Link/RConn1
  Pin/RConn1 -- Rev Pin/RConn1
  Rev Pin/LConn1 -- Inner Link/RConn2
  Pin/LConn1 -- Outer Link/RConn2

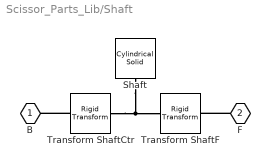
== system Scissor_Parts_Lib/Shaft ==
  Shaft : sm_lib/Body Elements/Cylindrical Solid  CylinderRadius=r  CylinderRadiusUnits=cm  CylinderLength=L  CylinderLengthUnits=cm  ExportEntireGeometry=off  InertiaType=CalculateFromGeometry  BasedOnType=Density  Density=Ro  DensityUnits=kg/m^3  Mass=1  MassUnits=kg  CenterOfMass=[0 0 0]  CenterOfMassUnits=m  MomentsOfInertia=[1 1 1]  MomentsOfInertiaUnits=kg*m^2  ProductsOfInertia=[0 0 0]  ProductsOfInertiaUnits=kg*m^2  GraphicType=FromGeometry  MarkerShape=Sphere  MarkerSize=1  GraphicVisPropType=SimpleVisualProperties  GraphicDiffuseColor=clr  GraphicOpacity=opc  GraphicSpecularColor=[0.2 0.2 0.2]  GraphicAmbientColor=[0.5 0.5 0.5]  GraphicEmissiveColor=[0.1 0.1 0.1]  GraphicShininess=24.0  DoExposeReferenceFrame=on  SerializedFrames=<Frames/>
  Transform ShaftCtr : sm_lib/Frames and Transforms/Rigid Transform  RotationMethod=StandardAxis  FollAlignAxisA=+X  BaseAlignAxisA=+Y  FollAlignAxisB=+Y  BaseAlignAxisB=+Z  RotationStandardAxis=+Z  RotationAngle=theta  RotationAngleUnits=deg  RotationArbitraryAxis=[0 0 1]  RotationSequenceAxes=FollowerAxes  RotationSequence=XYX  RotationSequenceAngles=[0 0 0]  RotationSequenceAnglesUnits=deg  RotationMatrix=[1 0 0; 0 1 0; 0 0 1]  Quaternion=[1 0 0 0]  TranslationMethod=Cartesian  TranslationCartesianOffset=[0 0 L/2]*z_ori  TranslationCartesianOffsetUnits=cm  TranslationStandardAxis=+Z  TranslationStandardOffset=0  TranslationStandardOffsetUnits=cm  TranslationROffset=0  TranslationROffsetUnits=m  TranslationThetaOffset=0  TranslationThetaOffsetUnits=deg  TranslationZOffset=0  TranslationZOffsetUnits=m
  Transform ShaftF : sm_lib/Frames and Transforms/Rigid Transform  RotationMethod=None  FollAlignAxisA=+X  BaseAlignAxisA=+Y  FollAlignAxisB=+Y  BaseAlignAxisB=+Z  RotationStandardAxis=+Z  RotationAngle=0  RotationAngleUnits=deg  RotationArbitraryAxis=[0 0 1]  RotationSequenceAxes=FollowerAxes  RotationSequence=XYX  RotationSequenceAngles=[0 0 0]  RotationSequenceAnglesUnits=deg  RotationMatrix=[1 0 0; 0 1 0; 0 0 1]  Quaternion=[1 0 0 0]  TranslationMethod=Cartesian  TranslationCartesianOffset=[0 0 L/2]*z_ori  TranslationCartesianOffsetUnits=cm  TranslationStandardAxis=+Z  TranslationStandardOffset=0  TranslationStandardOffsetUnits=cm  TranslationROffset=0  TranslationROffsetUnits=m  TranslationThetaOffset=0  TranslationThetaOffsetUnits=deg  TranslationZOffset=0  TranslationZOffsetUnits=m
  B : PMIOPort  Side=Left
  F : PMIOPort  Port=2  Side=Right
  connections:
  Transform ShaftCtr/LConn1 -- B/RConn1
  F/RConn1 -- Transform ShaftF/RConn1
  Shaft/RConn1 -- Transform ShaftF/LConn1 -- Transform ShaftCtr/RConn1
